simulink model "Control"  (R2023b)
settings: Solver=VariableStepAuto  StartTime=0.0  StopTime=0.5  RelTol=1e-3
values from neighbouring files (symbols this model uses):
  f_v = 1.7086e-04    (= 0.00017086)    [Control0.m]
  i = 12    [Control0.m]    (also in Electromechanical_coupling0.m; Figure3_9.m; Figure4_1819.m)
  J = J_m+J_eq+J_L/(i^2)    (= 0.000140202493333)    [Control0.m]    (also in Electromechanical_coupling0.m; Figure3_9.m = 0.000114299715556)
  J_eq = 3.53416e-6    (= 3.53416e-06)    [Control0.m]    (also in Electromechanical_coupling0.m)
  J_L = 4530e-6    (= 0.00453)    [Control0.m]    (also in Electromechanical_coupling0.m)
  J_m = 105.21e-6    (= 0.00010521)    [Control0.m]    (also in Electromechanical_coupling0.m)
  J_total = J_m+J_eq+(1/(i^2)+miu/i)*J_L    (= 0.000143184743333)    [Control0.m]
  Jeq = 3.53416e-6    (= 3.53416e-06)    [Figure3_9.m]    (also in Figure4_1819.m = 0.000143184743333)
  JL = 800e-6    (= 0.0008)    [Figure3_9.m]    (also in Figure4_1819.m = 0.00453)
  Jm = 105.21e-6    (= 0.00010521)    [Figure3_9.m]    (also in Figure4_1819.m)
  K_t = 3/2 * P_n * phi_f    (= 0.28077)    [Control0.m]    (also in Electromechanical_coupling0.m)
  Kic = 2000    [Control0.m]    (also in Figure3_9.m)
  Kic_2 = R_s/L_q    (= 719.178082192)    [Control0.m]
  Kis = 10    [Control0.m]    (also in Figure3_9.m = 20)
  Kis_2 = 1/(3*TPWM*delta^2)    (= 92.5925925926)    [Control0.m]
  Kpc = 3    [Control0.m]    (also in Figure3_9.m)
  Kpc_2 = L_q/(3*TPWM)    (= 4.86666666667)    [Control0.m]
  Kps = 0.15    [Control0.m]    (also in Figure3_9.m = 0.2)
  Kps_2 = J_total/(3*TPWM*delta*K_t)    (= 0.283317589592)    [Control0.m]
  Kt = 3/2 * Pn * Flux    (= 0.28077)    [Figure3_9.m]    (also in Figure4_1819.m)
  L_d = 1.46e-3    (= 0.00146)    [Control0.m]    (also in Electromechanical_coupling0.m)
  L_q = L_d    (= 0.00146)    [Control0.m]    (also in Electromechanical_coupling0.m)
  miu = 0.0079    [Control0.m]    (also in Figure4_1819.m)
  NtoW = pi / 30    (= 0.10471975512)    [Control0.m]    (also in Electromechanical_coupling0.m)
  P_n = 14    [Control0.m]    (also in Electromechanical_coupling0.m)
  phi_f = 0.01337    [Control0.m]    (also in Electromechanical_coupling0.m)
  R_s = 1.05    [Control0.m]    (also in Electromechanical_coupling0.m)
  T_c0 = 0.0104    [Control0.m]
  TPWM = 1/10000    (= 0.0001)    [Control0.m]
  U_dc = 72    [Control0.m]
  WtoN = 30 / pi    (= 9.54929658551)    [Control0.m]    (also in Electromechanical_coupling0.m)
undefined symbols (not defined in the file or in its folder): fv, Tc0
libraries: spsStairGeneratorLib x20, slpidlib x15, spsDCVoltageSourceLib x5, spsUniversalBridgeLib x5, spsPermanentMagnetSynchronousMachineLib x5, spsSVPWMGenerator2LevelLib x5, sps_lib x1, simulink x1
(part 3 of 3)

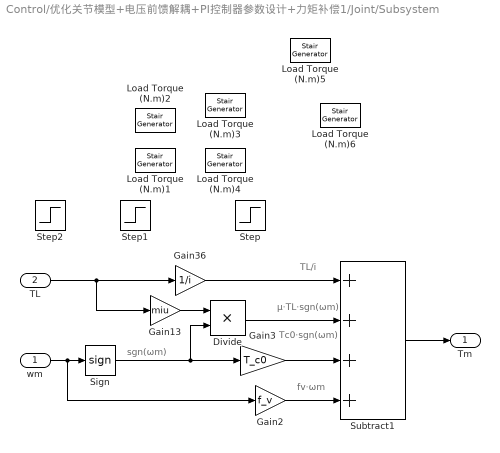
== system Control/优化关节模型+电压前馈解耦+PI控制器参数设计+力矩补偿1/Joint/Subsystem ==
  note: TL/i
  note: fv·ωm
  note: Tc0·sgn(ωm)
  note: μ·TL·sgn(ωm)
  note: sgn(ωm)
  wm : Inport
  TL : Inport  Port=2
  Divide : Product  Inputs=**
  Gain13 : Gain  Gain=miu
  Gain2 : Gain  Gain=f_v
  Gain3 : Gain  Gain=T_c0
  Gain36 : Gain  Gain=1/i
  Load Torque (N.m)1 : spsStairGeneratorLib/Stair Generator  t=[0,3,6,9,12,15,18,21,24]  e=[10,15,20,24.7,22.3,20.3,18.7,17.3,16.1]  Ts=1e-6
  Load Torque (N.m)2 : spsStairGeneratorLib/Stair Generator  t=[0,0.5,1,1.5,2.0,2.5,3,3.5,4]+0.2  e=[10,15,20,24.7,22.3,20.3,18.7,17.3,16.1]  Ts=1e-6
  Load Torque (N.m)3 : spsStairGeneratorLib/Stair Generator  t=[0 1.51 1.80 2.08 2.37 2.65]  e=[16.0,17.5,20,22.5,25,27.6]  Ts=1e-6
  Load Torque (N.m)4 : spsStairGeneratorLib/Stair Generator  t=[0 0.2 0.4 0.6 0.8 1 1.2 1.4 1.6 1.8 2 2.2]  e=[17 18 19 20 21 22 23 24 25 26 27.5 25]  Ts=1e-6
  Load Torque (N.m)5 : spsStairGeneratorLib/Stair Generator  t=[0,0.308,0.614,0.939,1.273,1.587,1.902,2.259,2.564]  e=[9.97,15,20,24.7,22.3,20.3,18.7,17.3,16.1]  Ts=1e-6
  Load Torque (N.m)6 : spsStairGeneratorLib/Stair Generator  t=[0 0.25 0.5 0.75 1 1.25 1.5 1.75 2]  e=[17 18 19 20 21 22 23 24 25]  Ts=1e-6
  Sign : Signum
  Step : Step  Time=0.3  After=2  SampleTime=0
  Step1 : Step  Time=0.3  Before=4  After=8  SampleTime=0
  Step2 : Step  Time=0.3  Before=4  After=6  SampleTime=0
  Subtract1 : Sum  Inputs=++++
  Tm : Outport
  wires:
  wm/1 -> Sign/1, Gain2/1
  Gain2/1 -> Subtract1/4
  Divide/1 -> Subtract1/2
  TL/1 -> Gain36/1, Gain13/1
  Sign/1 -> Gain3/1, Divide/2
  Gain13/1 -> Divide/1
  Gain3/1 -> Subtract1/3
  Subtract1/1 -> Tm/1
  Gain36/1 -> Subtract1/1

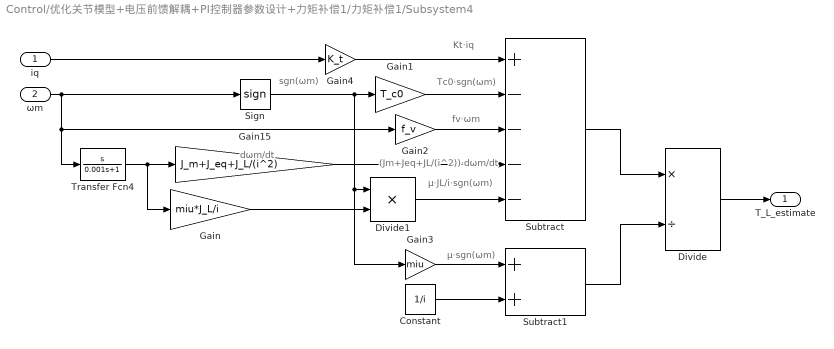
== system Control/优化关节模型+电压前馈解耦+PI控制器参数设计+力矩补偿1/力矩补偿1/Subsystem4 ==
  note: fv·ωm
  note: (Jm+Jeq+JL/(i^2))·dωm/dt
  note: Kt·iq
  note: Tc0·sgn(ωm)
  note: dωm/dt
  note: sgn(ωm)
  note: μ·JL/i·sgn(ωm)
  note: μ·sgn(ωm)
  iq : Inport
  ωm : Inport  Port=2
  Constant : Constant  Value=1/i
  Divide : Product  Inputs=*/
  Divide1 : Product  Inputs=**
  Gain : Gain  Gain=miu*J_L/i
  Gain1 : Gain  Gain=T_c0
  Gain15 : Gain  Gain=J_m+J_eq+J_L/(i^2)
  Gain2 : Gain  Gain=f_v
  Gain3 : Gain  Gain=miu
  Gain4 : Gain  Gain=K_t
  Sign : Signum
  Subtract : Sum  Inputs=+----
  Subtract1 : Sum
  Transfer Fcn4 : TransferFcn  Numerator=[1 0]  Denominator=[0.001 1]
  T_L_estimate : Outport
  wires:
  Gain4/1 -> Subtract/1
  ωm/1 -> Transfer Fcn4/1, Gain2/1, Sign/1
  Gain15/1 -> Subtract/4
  Divide/1 -> T_L_estimate/1
  Subtract/1 -> Divide/1
  Gain2/1 -> Subtract/3
  Gain1/1 -> Subtract/2
  Sign/1 -> Gain3/1, Divide1/1, Gain1/1
  iq/1 -> Gain4/1
  Constant/1 -> Subtract1/2
  Transfer Fcn4/1 -> Gain/1, Gain15/1
  Gain/1 -> Divide1/2
  Divide1/1 -> Subtract/5
  Gain3/1 -> Subtract1/1
  Subtract1/1 -> Divide/2

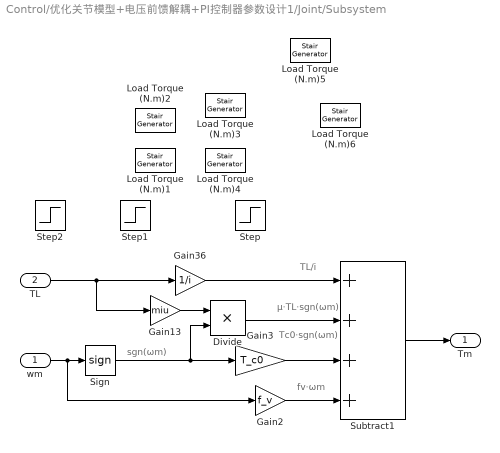
== system Control/优化关节模型+电压前馈解耦+PI控制器参数设计1/Joint/Subsystem ==
  note: sgn(ωm)
  note: μ·TL·sgn(ωm)
  note: Tc0·sgn(ωm)
  note: fv·ωm
  note: TL/i
  wm : Inport
  TL : Inport  Port=2
  Divide : Product  Inputs=**
  Gain13 : Gain  Gain=miu
  Gain2 : Gain  Gain=f_v
  Gain3 : Gain  Gain=T_c0
  Gain36 : Gain  Gain=1/i
  Load Torque (N.m)1 : spsStairGeneratorLib/Stair Generator  t=[0,3,6,9,12,15,18,21,24]  e=[10,15,20,24.7,22.3,20.3,18.7,17.3,16.1]  Ts=1e-6
  Load Torque (N.m)2 : spsStairGeneratorLib/Stair Generator  t=[0,0.5,1,1.5,2.0,2.5,3,3.5,4]+0.2  e=[10,15,20,24.7,22.3,20.3,18.7,17.3,16.1]  Ts=1e-6
  Load Torque (N.m)3 : spsStairGeneratorLib/Stair Generator  t=[0 1.51 1.80 2.08 2.37 2.65]  e=[16.0,17.5,20,22.5,25,27.6]  Ts=1e-6
  Load Torque (N.m)4 : spsStairGeneratorLib/Stair Generator  t=[0 0.2 0.4 0.6 0.8 1 1.2 1.4 1.6 1.8 2 2.2]  e=[17 18 19 20 21 22 23 24 25 26 27.5 25]  Ts=1e-6
  Load Torque (N.m)5 : spsStairGeneratorLib/Stair Generator  t=[0,0.308,0.614,0.939,1.273,1.587,1.902,2.259,2.564]  e=[9.97,15,20,24.7,22.3,20.3,18.7,17.3,16.1]  Ts=1e-6
  Load Torque (N.m)6 : spsStairGeneratorLib/Stair Generator  t=[0 0.25 0.5 0.75 1 1.25 1.5 1.75 2]  e=[17 18 19 20 21 22 23 24 25]  Ts=1e-6
  Sign : Signum
  Step : Step  Time=0.3  After=2  SampleTime=0
  Step1 : Step  Time=0.3  Before=4  After=8  SampleTime=0
  Step2 : Step  Time=0.3  Before=4  After=6  SampleTime=0
  Subtract1 : Sum  Inputs=++++
  Tm : Outport
  wires:
  Gain36/1 -> Subtract1/1
  Subtract1/1 -> Tm/1
  Gain3/1 -> Subtract1/3
  Gain13/1 -> Divide/1
  Sign/1 -> Divide/2, Gain3/1
  TL/1 -> Gain13/1, Gain36/1
  Divide/1 -> Subtract1/2
  Gain2/1 -> Subtract1/4
  wm/1 -> Gain2/1, Sign/1

== system Control/优化关节模型+电压前馈解耦1/Joint/Subsystem ==
  note: sgn(ωm)
  note: μ·TL·sgn(ωm)
  note: Tc0·sgn(ωm)
  note: fv·ωm
  note: TL/i
  wm : Inport
  TL : Inport  Port=2
  Divide : Product  Inputs=**
  Gain13 : Gain  Gain=miu
  Gain2 : Gain  Gain=f_v
  Gain3 : Gain  Gain=T_c0
  Gain36 : Gain  Gain=1/i
  Load Torque (N.m)3 : spsStairGeneratorLib/Stair Generator  t=[0 1.51 1.80 2.08 2.37 2.65]  e=[16.0,17.5,20,22.5,25,27.6]  Ts=1e-6
  Sign : Signum
  Subtract1 : Sum  Inputs=++++
  Tm : Outport
  wires:
  Gain36/1 -> Subtract1/1
  Subtract1/1 -> Tm/1
  Gain3/1 -> Subtract1/3
  Gain13/1 -> Divide/1
  Sign/1 -> Divide/2, Gain3/1
  TL/1 -> Gain13/1, Gain36/1
  Divide/1 -> Subtract1/2
  Gain2/1 -> Subtract1/4
  wm/1 -> Gain2/1, Sign/1

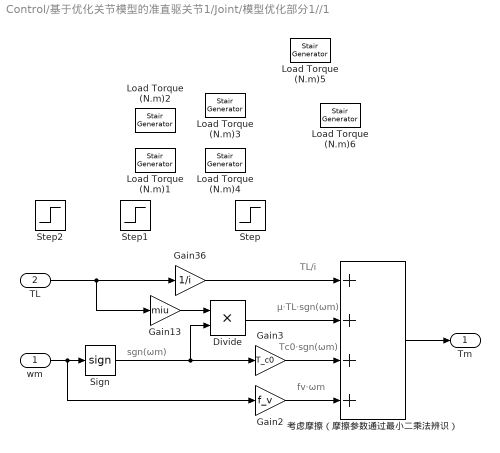
== system Control/基于优化关节模型的准直驱关节1/Joint/模型优化部分1//1 ==
  note: sgn(ωm)
  note: μ·TL·sgn(ωm)
  note: Tc0·sgn(ωm)
  note: fv·ωm
  note: TL/i
  wm : Inport
  TL : Inport  Port=2
  Divide : Product  Inputs=**
  Gain13 : Gain  Gain=miu
  Gain2 : Gain  Gain=f_v
  Gain3 : Gain  Gain=T_c0
  Gain36 : Gain  Gain=1/i
  Load Torque (N.m)1 : spsStairGeneratorLib/Stair Generator  t=[0,3,6,9,12,15,18,21,24]  e=[10,15,20,24.7,22.3,20.3,18.7,17.3,16.1]  Ts=1e-6
  Load Torque (N.m)2 : spsStairGeneratorLib/Stair Generator  t=[0,0.5,1,1.5,2.0,2.5,3,3.5,4]+0.2  e=[10,15,20,24.7,22.3,20.3,18.7,17.3,16.1]  Ts=1e-6
  Load Torque (N.m)3 : spsStairGeneratorLib/Stair Generator  t=[0 1.51 1.80 2.08 2.37 2.65]  e=[16.0,17.5,20,22.5,25,27.6]  Ts=1e-6
  Load Torque (N.m)4 : spsStairGeneratorLib/Stair Generator  t=[0 0.2 0.4 0.6 0.8 1 1.2 1.4 1.6 1.8 2 2.2]  e=[17 18 19 20 21 22 23 24 25 26 27.5 25]  Ts=1e-6
  Load Torque (N.m)5 : spsStairGeneratorLib/Stair Generator  t=[0,0.308,0.614,0.939,1.273,1.587,1.902,2.259,2.564]  e=[9.97,15,20,24.7,22.3,20.3,18.7,17.3,16.1]  Ts=1e-6
  Load Torque (N.m)6 : spsStairGeneratorLib/Stair Generator  t=[0 0.25 0.5 0.75 1 1.25 1.5 1.75 2]  e=[17 18 19 20 21 22 23 24 25]  Ts=1e-6
  Sign : Signum
  Step : Step  Time=0.3  After=2  SampleTime=0
  Step1 : Step  Time=0.3  Before=4  After=8  SampleTime=0
  Step2 : Step  Time=0.3  Before=4  After=6  SampleTime=0
  考虑摩擦（摩擦参数通过最小二乘法辨识） : Sum  Inputs=++++
  Tm : Outport
  wires:
  Gain36/1 -> 考虑摩擦（摩擦参数通过最小二乘法辨识）/1
  考虑摩擦（摩擦参数通过最小二乘法辨识）/1 -> Tm/1
  Gain3/1 -> 考虑摩擦（摩擦参数通过最小二乘法辨识）/3
  Gain13/1 -> Divide/1
  Sign/1 -> Divide/2, Gain3/1
  TL/1 -> Gain13/1, Gain36/1
  Divide/1 -> 考虑摩擦（摩擦参数通过最小二乘法辨识）/2
  Gain2/1 -> 考虑摩擦（摩擦参数通过最小二乘法辨识）/4
  wm/1 -> Gain2/1, Sign/1

== matlab function Control/优化关节模型+电压前馈解耦1/反Park变换 ==
  data: u_d input; u_q input; u_alpha output; u_beta output; theta_e input
function [u_alpha, u_beta]  = inv_park(u_d,u_q,theta_e)

u_alpha=cos(theta_e)*u_d-sin(theta_e)*u_q;
u_beta=sin(theta_e)*u_d+cos(theta_e)*u_q;

end

== matlab function Control/优化关节模型+电压前馈解耦+PI控制器参数设计1/MATLAB Function3 ==
  data: i_a input; i_alpha output; i_b input; i_c input; i_beta output
function [i_alpha, i_beta] = clarke(i_a,i_b,i_c)

i_alpha=(i_a-1/2*i_b-1/2*i_c)*2/3;
i_beta=(sqrt(3)/2*i_b-sqrt(3)/2*i_c)*2/3;

== matlab function Control/优化关节模型+电压前馈解耦+PI控制器参数设计1/MATLAB Function4 ==
  data: i_d output; i_q output; i_alpha input; i_beta input; theta_e input
function [i_d,i_q] = park(i_alpha,i_beta,theta_e)

i_d=i_alpha*cos(theta_e)+i_beta*sin(theta_e);
i_q=-i_alpha*sin(theta_e)+i_beta*cos(theta_e);
% I_d=-(I_alph.*cos(theta)+I_beta.*sin(theta));
% I_q= -(-I_alph.*sin(theta)+I_beta.*cos(theta));

== matlab function Control/优化关节模型+电压前馈解耦+PI控制器参数设计1/反Park变换 ==
  data: u_d input; u_q input; u_alpha output; u_beta output; theta_e input
function [u_alpha, u_beta]  = inv_park(u_d,u_q,theta_e)

u_alpha=cos(theta_e)*u_d-sin(theta_e)*u_q;
u_beta=sin(theta_e)*u_d+cos(theta_e)*u_q;

end

== matlab function Control/优化关节模型+电压前馈解耦+PI控制器参数设计+力矩补偿1/MATLAB Function3 ==
  data: i_a input; i_alpha output; i_b input; i_c input; i_beta output
function [i_alpha, i_beta] = clarke(i_a,i_b,i_c)

i_alpha=(i_a-1/2*i_b-1/2*i_c)*2/3;
i_beta=(sqrt(3)/2*i_b-sqrt(3)/2*i_c)*2/3;

== matlab function Control/优化关节模型+电压前馈解耦+PI控制器参数设计+力矩补偿1/MATLAB Function4 ==
  data: i_d output; i_q output; i_alpha input; i_beta input; theta_e input
function [i_d,i_q] = park(i_alpha,i_beta,theta_e)

i_d=i_alpha*cos(theta_e)+i_beta*sin(theta_e);
i_q=-i_alpha*sin(theta_e)+i_beta*cos(theta_e);
% I_d=-(I_alph.*cos(theta)+I_beta.*sin(theta));
% I_q= -(-I_alph.*sin(theta)+I_beta.*cos(theta));

== matlab function Control/理想关节模型1/ABC计算及扇区判断 ==
  data: u_alpha input; X output; Y output; Z output; u_beta input; N output; U_dc input; T input
%% 计算ABC的值，用于计算N值，以判断扇区
function [X,Y,Z,N] = fcn(u_alpha,u_beta,U_dc,T)
%--------------------为了方便推导作用时间做出的设定值------------------------
X=(sqrt(3)*T/U_dc)*u_beta;                           
Y=(sqrt(3)*T/U_dc)*(sqrt(3)/2*u_alpha+1/2*u_beta);     
Z=(sqrt(3)*T/U_dc)*(-sqrt(3)/2*u_alpha+1/2*u_beta);      
%--------------------------------扇区值判断---------------------------------
%Uref1*sqrt(3)
%(Uref1+Uref2)*sqrt(3)
%(Uref1+Uref3)*sqrt(3)
%--------------------------------------------------------------------------
u_refA=u_beta;
u_refB=(sqrt(3)*u_alpha/2-u_beta/2);
u_refC=(-sqrt(3)*u_alpha/2-u_beta/2);
if(u_refA>0)                                       %Uref1>0
    A=1;
else
    A=0;
end                                                                                                                                                                                                                                                                                                                                                                                                                                                                                                                                                                                                                                                                                                                                                                                                                                                                                                                                                                                                                                                                                                                                                                                                                                                                                   
if(u_refB>0)                     %Uref2>0
    B=1;
else
    B=0; 
end
if(u_refC>0)                    %%Uref3>0
    C=1;
else
    C=0;
end
N=A+2*B+4*C;

== matlab function Control/优化关节模型+电压前馈解耦+PI控制器参数设计+力矩补偿1/反Park变换 ==
  data: u_d input; u_q input; u_alpha output; u_beta output; theta_e input
function [u_alpha, u_beta]  = inv_park(u_d,u_q,theta_e)

u_alpha=cos(theta_e)*u_d-sin(theta_e)*u_q;
u_beta=sin(theta_e)*u_d+cos(theta_e)*u_q;

end

== matlab function Control/理想关节模型1/MATLAB Function3 ==
  data: i_a input; i_alpha output; i_b input; i_c input; i_beta output
function [i_alpha, i_beta] = clarke(i_a,i_b,i_c)

i_alpha=(i_a-1/2*i_b-1/2*i_c)*2/3;
i_beta=(sqrt(3)/2*i_b-sqrt(3)/2*i_c)*2/3;

== matlab function Control/理想关节模型1/MATLAB Function4 ==
  data: i_q output; i_alpha input; i_d output; i_beta input; theta_e input
function [i_q,i_d] = park(i_alpha,i_beta,theta_e)

i_d=i_alpha*cos(theta_e)+i_beta*sin(theta_e);
i_q=-i_alpha*sin(theta_e)+i_beta*cos(theta_e);
% I_d=-(I_alph.*cos(theta)+I_beta.*sin(theta));
% I_q= -(-I_alph.*sin(theta)+I_beta.*cos(theta));

== matlab function Control/理想关节模型1/反Park变换 ==
  data: u_d input; u_q input; u_alpha output; u_beta output; theta_e input
function [u_alpha, u_beta]  = inv_park(u_d,u_q,theta_e)

u_alpha=cos(theta_e)*u_d-sin(theta_e)*u_q;
u_beta=sin(theta_e)*u_d+cos(theta_e)*u_q;

end

== matlab function Control/理想关节模型1/切换时间计算 ==
  data: T_first input; Tcm1 output; T_second input; T_0 input; N input; Tcm2 output; Tcm3 output
function [Tcm1,Tcm2,Tcm3] = fcn(T_first,T_second,T_0,N)

T_a=T_0/2.0;
T_b=T_a+T_first/2.0;
T_c=T_b+T_second/2.0;

switch N
    case 1 %% 扇区II
        Tcm1=T_b;
        Tcm2=T_a;
        Tcm3=T_c;
    case 2  %% 扇区VI
        Tcm1=T_a;
        Tcm2=T_c;
        Tcm3=T_b;
    case 3  %% 扇区I
        Tcm1=T_a;
        Tcm2=T_b;
        Tcm3=T_c;
    case 4  %% 扇区IV
        Tcm1=T_c;
        Tcm2=T_b;
        Tcm3=T_a;
    case 5  %% 扇区III
        Tcm1=T_c;
        Tcm2=T_a;
        Tcm3=T_b;
    otherwise %% 扇区V
        Tcm1=T_b;
        Tcm2=T_c;
        Tcm3=T_a;
end

== matlab function Control/理想关节模型1/矢量作用时间计算 ==
  data: X input; T_first output; Y input; Z input; N input; T_second output; T_0 output; T input; N output
function [T_first,T_second,T_0,N] = fcn(X,Y,Z,N,T) 
switch(N)
    case 1
        S=2;%----------------------扇区编号S---------------------------
        T_first=Z; 
        T_second=Y; 
    case 2
        S=6;
        T_first=Y; 
        T_second=-X;
    case 3
        S=1;
        T_first=-Z; 
        T_second=X;
    case 4
        S=4;
        T_first=-X; 
        T_second=Z;
    case 5
        S=3;
        T_first=X; 
        T_second=-Y;
    case 6
        S=5;
        T_first=-Y; 
        T_second=-Z;
    otherwise
        S=1;
        T_first=0; 
        T_second=0;        
end
%--------------------------------------------------------------------------
%-----------------------------是否需要调制判断------------------------------
if((T_first+T_second)>T)
    t11=T_first*T/(T_first+T_second);
    t21=T_second*T/(T_first+T_second);
    T_first=t11;
    T_second=t21;
    T_0=0;
else
T_0=(T-T_first-T_second)/2;
end

== matlab function Control/基于优化关节模型的准直驱关节1/MATLAB Function3 ==
  data: i_a input; i_alpha output; i_b input; i_c input; i_beta output
function [i_alpha, i_beta] = clarke(i_a,i_b,i_c)

i_alpha=(i_a-1/2*i_b-1/2*i_c)*2/3;
i_beta=(sqrt(3)/2*i_b-sqrt(3)/2*i_c)*2/3;

== matlab function Control/基于优化关节模型的准直驱关节1/MATLAB Function4 ==
  data: i_q output; i_alpha input; i_d output; i_beta input; theta_e input
function [i_q,i_d] = park(i_alpha,i_beta,theta_e)

i_d=i_alpha*cos(theta_e)+i_beta*sin(theta_e);
i_q=-i_alpha*sin(theta_e)+i_beta*cos(theta_e);
% I_d=-(I_alph.*cos(theta)+I_beta.*sin(theta));
% I_q= -(-I_alph.*sin(theta)+I_beta.*cos(theta));

== matlab function Control/基于优化关节模型的准直驱关节1/反Park变换 ==
  data: u_d input; u_q input; u_alpha output; u_beta output; theta_e input
function [u_alpha, u_beta]  = inv_park(u_d,u_q,theta_e)

u_alpha=cos(theta_e)*u_d-sin(theta_e)*u_q;
u_beta=sin(theta_e)*u_d+cos(theta_e)*u_q;

end

== matlab function Control/优化关节模型+电压前馈解耦1/MATLAB Function3 ==
  data: i_a input; i_alpha output; i_b input; i_c input; i_beta output
function [i_alpha, i_beta] = clarke(i_a,i_b,i_c)

i_alpha=(i_a-1/2*i_b-1/2*i_c)*2/3;
i_beta=(sqrt(3)/2*i_b-sqrt(3)/2*i_c)*2/3;

== matlab function Control/优化关节模型+电压前馈解耦1/MATLAB Function4 ==
  data: i_d output; i_q output; i_alpha input; i_beta input; theta_e input
function [i_d,i_q] = park(i_alpha,i_beta,theta_e)

i_d=i_alpha*cos(theta_e)+i_beta*sin(theta_e);
i_q=-i_alpha*sin(theta_e)+i_beta*cos(theta_e);
% I_d=-(I_alph.*cos(theta)+I_beta.*sin(theta));
% I_q= -(-I_alph.*sin(theta)+I_beta.*cos(theta));
